simulink model "inv_psm"  (R2026b)
settings: Solver=ode23tb  StopTime=param.sim.simlength  FixedStep=param.sim.tc  MaxStep=param.glb_time.tc
values from neighbouring files (symbols this model uses):
  param = struct()    [init_model.m]
undefined symbols (not defined in the file or in its folder): magnitude
libraries: fl_lib x155, nesl_utility x77, igbt_simple_2th_lib x6, lithium_ion_battery x2, simple_flexible_shaft x2, cstblocks_lti x2, dclink_with_center_tap x1, three_phase_pwm_modulator x1, three_phase_inverter_ideal_switch_based_model x1, three_phase_inverter_igbt_advanced_thermal_model x1, three_phase_inverter_mosfet_based_with_thermal_model x1, threephase_inductor_lib x1
(part 1 of 6)
settings Model: Creator=dbagn  LastModifiedBy=dbagn
settings SolverCC: SolverResetMethod=Robust  ZeroCrossControl=DisableAll
settings DataIOCC: DSMLogging=off  ReturnWorkspaceOutputs=off  SaveOutput=off  SaveTime=off  SignalLogging=off
settings OptimizationCC: ReuseModelBlockBuffer=off
settings SFSimCC: CustomCodeUndefinedFunction=ThrowError  DefaultCustomCodeDeterministicFunctions=All
settings SFSimCC: SimCustomHeaderCode=|
  | #include "rpi.h"
  | #include "mavgflt.h"
  | #include "mavgflt_simulink.h"
  | #include "mavgflts.h"
  | #include "mavgflts_simulink.h"
  | #include "dsmavgflt.h"
  | #include "dsmavgflt_simulink.h"
  | #include "bemf_obsv.h"
  | #include "bemf_obsv_simulink.h"
  | #include "bemf_obsv_load_est.h"
  | #include "bemf_obsv_load_est_simulink.h"
  | #include "dqvector_pi.h"
  | #include "dqvector_pi_simulink.h"
  | #include "sv_pwm_simulink.h"
  | #include "sv_pwm.h"
  | #include "first_harmonic_tracker.h"
  | #include "first_harmonic_tracker_simulink.h"
  | #include "dqpll_thyr.h"
  | #include "dqpll_thyr_simulink.h"
  | #include "dqpll_grid.h"
  | #include "dqpll_grid_simulink.h"
settings SFSimCC: SimUserIncludeDirs=|
  | include
  | src
settings SFSimCC: SimUserSources=|
  | "rpi.c"
  | "mavgflt_simulink.c"
  | "mavgflt.c"
  | "mavgflts_simulink.c"
  | "mavgflts.c"
  | "dsmavgflt_simulink.c"
  | "dsmavgflt.c"
  | "bemf_obsv_simulink.c"
  | "bemf_obsv.c"
  | "bemf_obsv_load_est_simulink.c"
  | "bemf_obsv_load_est.c"
  | "dqvector_pi.c"
  | "dqvector_pi_simulink.c"
  | "sv_pwm_simulink.c"
  | "sv_pwm.c"
  | "first_harmonic_tracker_simulink.c"
  | "first_harmonic_tracker.c"
  | "dqpll_thyr_simulink.c"
  | "dqpll_thyr.c"
  | "dqpll_grid_simulink.c"
  | "dqpll_grid.c"
settings RTWCC: DLArmComputeVersion=19.05
settings SimscapeCC: SimscapeUseEnergyAccounting=off

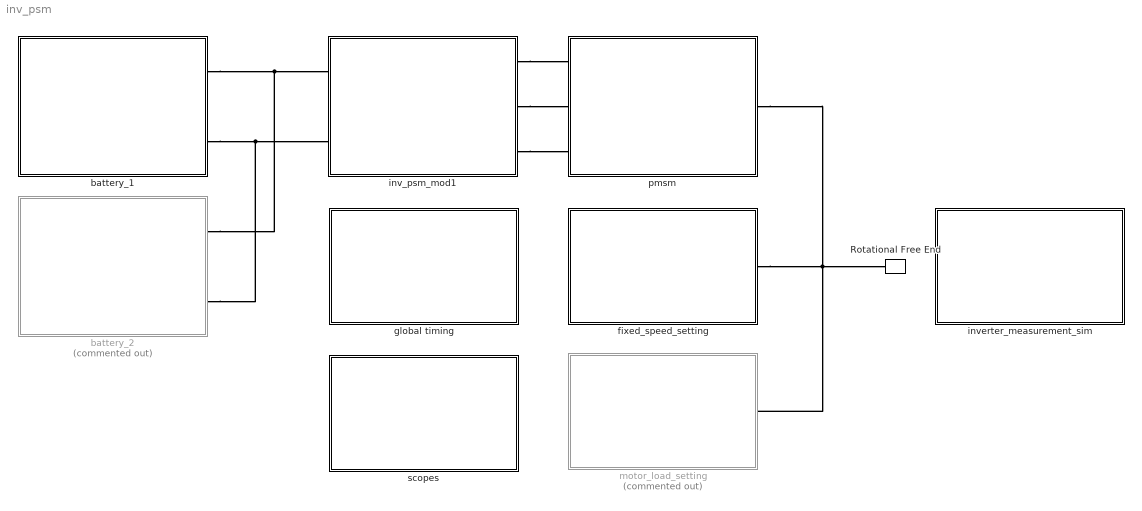
== system inv_psm ==
  Rotational Free End : fl_lib/Mechanical/Rotational Elements/Rotational Free End  w_specify=off  w_priority=None  w=0 rad/s  w_nominal_specify=off  w_nominal_value=1  w_nominal_unit=rad/s
  battery_1 : Subsystem
  battery_2 : Subsystem  Commented=on
  fixed_speed_setting : Subsystem
  global timing : Subsystem
  inv_psm_mod1 : Subsystem
  inverter_measurement_sim : Subsystem
  motor_load_setting : Subsystem  Commented=on
  pmsm : Subsystem
  scopes : Subsystem
  connections:
  pmsm/RConn1 -- Rotational Free End/LConn1 -- fixed_speed_setting/LConn1 -- motor_load_setting/LConn1
  inv_psm_mod1/RConn2 -- pmsm/LConn2
  inv_psm_mod1/RConn1 -- pmsm/LConn1
  inv_psm_mod1/RConn3 -- pmsm/LConn3
  battery_1/RConn1 -- battery_2/RConn1 -- inv_psm_mod1/LConn1
  battery_1/RConn2 -- inv_psm_mod1/LConn2 -- battery_2/RConn2

== system inv_psm/battery_1 ==
  Solver Configuration1 : nesl_utility/Solver Configuration  PhysicalDomain=network_engine_domain  SubClassName=solver  LeftPortType=input  RightPortType=generic  Tones=[]  Harmonics=[]  SimulateNoise=off  Profile=off  UseLocalSampling=off  EnableSwitchedLinearOptims=on  FrequencyDomain=off  UseCCode=off  RelTol=0.001  AbsTol=0.001  MinStep=1e-09  ToWorkspace=off  RevertToSquareIcSolve=off  NumHomotopyIterations=100  PhasorMode=off  PhasorModeNumHarmonics=1  ConsistencySolver=NEWTON_XTOL_AFTER_FTOL  CanonicalOrdering=CANONICAL  OptimizeIntermediates=OPTIMIZED  MulticoreSolverChoice=BACKWARD_EULER  IndexReductionMethod=DerivativeReplacement  DoDC=on  ResidualTolerance=1e-09  ConsistencyTolSource=GLOBAL  ConsistencyAbsTol=0.001  ConsistencyRelTol=0.001  ConsistencyTolFactor=0.001  UseLocalSolver=on  LocalSolverChoice=NE_BACKWARD_EULER_ADVANCER  ResolveIndetEquations=on  FunctionEvalNumThread=1  LocalSolverSampleTime=param.glb_time.tc  DoFixedCost=on  MaxNonlinIter=param.sim.nonlinear_iterations  MaxModeIter=2  ComputeImpulses=off  ImpulseIterations=2  LinearAlgebra=auto  LinearAlgebraNumThread=0  EquationFormulation=NE_TIME_EF  DelaysMemoryBudget=1024  AutomaticFiltering=on  FilteringTimeConstant=0.001  PartitionStorageMethod=AS_NEEDED  PartitionMemoryBudget=1024  PartitionMethod=BALANCED  MultibodyUseLocalSolver=off  MultibodyLocalSolverChoice=ODE1  MultibodyLocalSolverSampleTime=0.001
  litium ion battery 1 : Scope
      settings: ActiveDisplayYMinimum=-166.63080014270002  ActiveDisplayYMaximum=1499.6922306374129  DataLoggingVariableName=ScopeData3
  litium_ion_battery : lithium_ion_battery/lithium_ion_battery  Q=param.battery.pack_1.Q  number_of_cells=param.battery.pack_1.number_of_cells  E_1=param.battery.pack_1.E_1  E0=param.battery.pack_1.E0  E1=param.battery.pack_1.E1  E2=param.battery.pack_1.E2  E3=param.battery.pack_1.E3  Elog=param.battery.pack_1.Elog  R0=param.battery.pack_1.R0  R1=param.battery.pack_1.R1  C1=param.battery.pack_1.C1  M=param.battery.pack_1.M  alpha=param.battery.pack_1.alpha  soc_init=param.battery.pack_1.soc_init  ts_battery=param.glb_time.ts_dab  q1Kalman=param.battery.pack_1.q1Kalman  q2Kalman=param.battery.pack_1.q2Kalman  q3Kalman=param.battery.pack_1.q3Kalman  rKalman=param.battery.pack_1.rKalman  tc=param.glb_time.tc  enable_white_noise_m=0  battery_voltage_init_m=param.battery.nominal_battery_voltage_1
  single_phase_ui_measure : Subsystem
  dc+ : PMIOPort  Side=Right
  dc- : PMIOPort  Port=2  Side=Right
  wires:
  litium_ion_battery/1 -> litium ion battery 1/1
  connections:
  single_phase_ui_measure/LConn2 -- Solver Configuration1/RConn1 -- litium_ion_battery/RConn2
  single_phase_ui_measure/RConn1 -- dc+/RConn1
  litium_ion_battery/RConn1 -- single_phase_ui_measure/LConn1
  dc-/RConn1 -- single_phase_ui_measure/RConn2

== system inv_psm/battery_2 ==
  litium ion battery 2 : Scope
      settings: ActiveDisplayYMinimum=-4779.68523514888  ActiveDisplayYMaximum=38953.418417165572  DataLoggingVariableName=ScopeData3
  litium_ion_battery : lithium_ion_battery/lithium_ion_battery  Q=param.battery.pack_2.Q  number_of_cells=param.battery.pack_2.number_of_cells  E_1=param.battery.pack_2.E_1  E0=param.battery.pack_2.E0  E1=param.battery.pack_2.E1  E2=param.battery.pack_2.E2  E3=param.battery.pack_2.E3  Elog=param.battery.pack_2.Elog  R0=param.battery.pack_2.R0  R1=param.battery.pack_2.R1  C1=param.battery.pack_2.C1  M=param.battery.pack_2.M  alpha=param.battery.pack_2.alpha  soc_init=param.battery.pack_2.soc_init  ts_battery=param.glb_time.ts_dab  q1Kalman=param.battery.pack_2.q1Kalman  q2Kalman=param.battery.pack_2.q2Kalman  q3Kalman=param.battery.pack_2.q3Kalman  rKalman=param.battery.pack_2.rKalman  tc=param.glb_time.tc  enable_white_noise_m=0  battery_voltage_init_m=param.battery.nominal_battery_voltage_1
  single_phase_ui_measure : Subsystem
  dc+ : PMIOPort  Side=Right
  dc- : PMIOPort  Port=2  Side=Right
  wires:
  litium_ion_battery/1 -> litium ion battery 2/1
  connections:
  dc-/RConn1 -- single_phase_ui_measure/RConn2
  litium_ion_battery/RConn1 -- single_phase_ui_measure/LConn1
  single_phase_ui_measure/RConn1 -- dc+/RConn1
  single_phase_ui_measure/LConn2 -- litium_ion_battery/RConn2

== system inv_psm/fixed_speed_setting ==
  Ideal Angular Velocity Source : fl_lib/Mechanical/Mechanical Sources/Ideal Angular Velocity Source
  Mechanical Rotational Reference : fl_lib/Mechanical/Rotational Elements/Mechanical Rotational Reference
  PS Add : fl_lib/Physical Signals/Functions/PS Add
  PS Step1 : fl_lib/Physical Signals/Sources/PS Step  step_time=0.025 s  initial_value=0 rpm  final_value=param.load.rpm_sim rpm
  PS Step2 : fl_lib/Physical Signals/Sources/PS Step  step_time=1.0 s  initial_value=0 rpm  final_value=-2*param.load.rpm_sim rpm
  PS Transfer Function : fl_lib/Physical Signals/Linear Operators/PS Transfer Function  transfer_function_type=foundation.enum.transfer_function_type.lag  T=0.25 s  T1=2 s  T2=1 s  reset_method=foundation.enum.IntegratorResetSpec.None  initial_condition_spec=foundation.enum.IntegratorICSpec.Internal  y0=0 rpm
  flexible_shaft : simple_flexible_shaft/flexible_shaft  Commented=through  b1=1  b2=1  J1=1  J2=1  b_displacement=1e5  k_displacement=1e8
  shaft : PMIOPort  Side=Left
  connections:
  Mechanical Rotational Reference/LConn1 -- Ideal Angular Velocity Source/RConn2
  PS Transfer Function/RConn1 -- Ideal Angular Velocity Source/RConn1
  shaft/RConn1 -- flexible_shaft/LConn1
  flexible_shaft/RConn1 -- Ideal Angular Velocity Source/LConn1
  PS Add/LConn1 -- PS Step1/RConn1
  PS Add/LConn2 -- PS Step2/RConn1
  PS Add/RConn1 -- PS Transfer Function/LConn1

== system inv_psm/global timing ==
  From9 : From  Commented=on  GotoTag=local_time_corr_afe1
  Unit Delay : UnitDelay  SampleTime=param.glb_time.tc
  Unit Delay1 : UnitDelay  SampleTime=param.glb_time.tc
  time_afe1 : Subsystem  mask{k=param.afe.behav.time_gain_module_1}
      mask prompts: k "Time Gain"
      mask Display:
      | disp('time-gen');
      | port_label('input', 1, 'crt');
      | port_label('output', 1, 'tout');
  time_afe3 : Subsystem  mask{k=1}
      mask prompts: k "Time Gain"
      mask Display:
      | disp('time-gen');
      | port_label('output', 1, 'tout');
  time_inv1 : Subsystem  mask{k=param.inv.behav.time_gain_module_2}
      mask prompts: k "Time Gain"
      mask Display:
      | disp('time-gen');
      | port_label('input', 1, 'crt');
      | port_label('output', 1, 'tout');
  tag scope: time_afe_module_1=global, time_inv_module_1=global, time_master=global
  wires:
  time_afe1/1(Out1) -> [time_afe_module_1]
  time_inv1/1(Out1) -> [time_inv_module_1]
  time_afe3/1(Out1) -> [time_master]
  Unit Delay/1 -> time_afe1/1(correction_time)
  Unit Delay1/1 -> time_inv1/1(correction_time)

== system inv_psm/inv_psm_mod1 ==
  dc_source : Subsystem
  inverter : Subsystem
  inverter_ctrl : Subsystem
  output_filter : Subsystem
  us_u : PMIOPort  Side=Right
  us_v : PMIOPort  Port=2  Side=Right
  us_w : PMIOPort  Port=3  Side=Right
  udc(+) : PMIOPort  Port=4  Side=Left
  udc(-) : PMIOPort  Port=5  Side=Left
  wires:
  inverter_ctrl/1(duvw_out) -> inverter/1(duvw)
  connections:
  inverter/LConn2 -- output_filter/RConn2
  inverter/LConn1 -- output_filter/RConn1
  inverter/LConn3 -- output_filter/RConn3
  output_filter/LConn2 -- us_v/RConn1
  output_filter/LConn3 -- us_w/RConn1
  output_filter/LConn1 -- us_u/RConn1
  inverter/RConn1 -- dc_source/RConn1
  inverter/RConn2 -- dc_source/RConn2
  dc_source/LConn2 -- udc(-)/RConn1
  dc_source/LConn1 -- udc(+)/RConn1

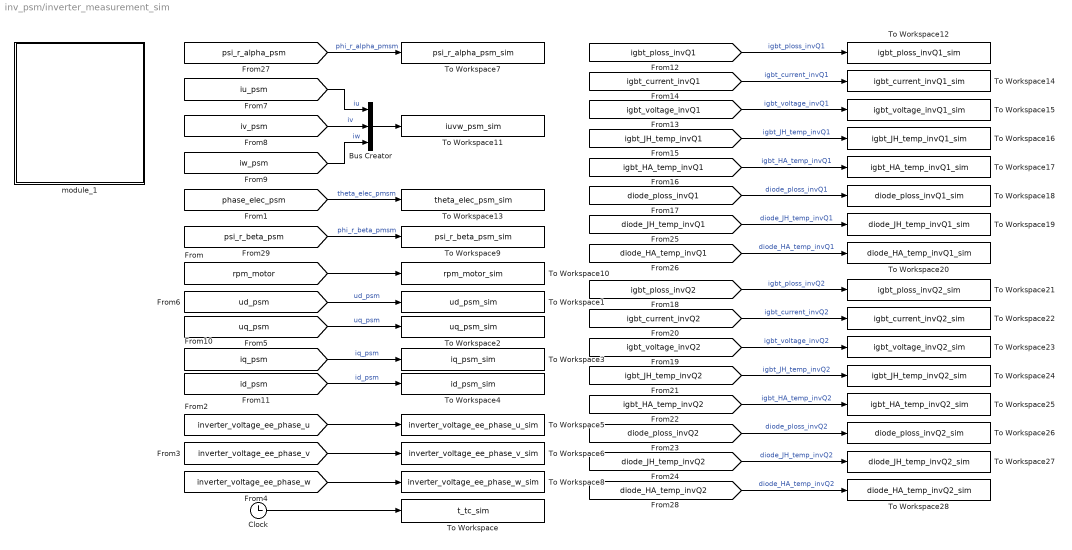
== system inv_psm/inverter_measurement_sim ==
  Bus Creator : BusCreator  Inputs=3
  Clock : Clock
  To Workspace : ToWorkspace  VariableName=t_tc_sim  SampleTime=param.glb_time.tc
      settings: MaxDataPoints=param.glb_time.Nc  Decimation=param.glb_time.decimation_tc
  To Workspace1 : ToWorkspace  VariableName=ud_psm_sim  SampleTime=param.glb_time.tc
      settings: MaxDataPoints=param.glb_time.Nc  Decimation=param.glb_time.decimation_tc
  To Workspace10 : ToWorkspace  VariableName=rpm_motor_sim  SampleTime=param.glb_time.tc
      settings: MaxDataPoints=param.glb_time.Nc  Decimation=param.glb_time.decimation_tc
  To Workspace11 : ToWorkspace  VariableName=iuvw_psm_sim  SampleTime=param.glb_time.tc
      settings: MaxDataPoints=param.glb_time.Nc  Decimation=param.glb_time.decimation_tc
  To Workspace12 : ToWorkspace  VariableName=igbt_ploss_invQ1_sim  SampleTime=param.glb_time.tc
      settings: MaxDataPoints=param.glb_time.Nc  Decimation=param.glb_time.decimation_tc
  To Workspace13 : ToWorkspace  VariableName=theta_elec_psm_sim  SampleTime=param.glb_time.tc
      settings: MaxDataPoints=param.glb_time.Nc  Decimation=param.glb_time.decimation_tc
  To Workspace14 : ToWorkspace  VariableName=igbt_current_invQ1_sim  SampleTime=param.glb_time.tc
      settings: MaxDataPoints=param.glb_time.Nc  Decimation=param.glb_time.decimation_tc
  To Workspace15 : ToWorkspace  VariableName=igbt_voltage_invQ1_sim  SampleTime=param.glb_time.tc
      settings: MaxDataPoints=param.glb_time.Nc  Decimation=param.glb_time.decimation_tc
  To Workspace16 : ToWorkspace  VariableName=igbt_JH_temp_invQ1_sim  SampleTime=param.glb_time.tc
      settings: MaxDataPoints=param.glb_time.Nc  Decimation=param.glb_time.decimation_tc
  To Workspace17 : ToWorkspace  VariableName=igbt_HA_temp_invQ1_sim  SampleTime=param.glb_time.tc
      settings: MaxDataPoints=param.glb_time.Nc  Decimation=param.glb_time.decimation_tc
  To Workspace18 : ToWorkspace  VariableName=diode_ploss_invQ1_sim  SampleTime=param.glb_time.tc
      settings: MaxDataPoints=param.glb_time.Nc  Decimation=param.glb_time.decimation_tc
  To Workspace19 : ToWorkspace  VariableName=diode_JH_temp_invQ1_sim  SampleTime=param.glb_time.tc
      settings: MaxDataPoints=param.glb_time.Nc  Decimation=param.glb_time.decimation_tc
  To Workspace2 : ToWorkspace  VariableName=uq_psm_sim  SampleTime=param.glb_time.tc
      settings: MaxDataPoints=param.glb_time.Nc  Decimation=param.glb_time.decimation_tc
  To Workspace20 : ToWorkspace  VariableName=diode_HA_temp_invQ1_sim  SampleTime=param.glb_time.tc
      settings: MaxDataPoints=param.glb_time.Nc  Decimation=param.glb_time.decimation_tc
  To Workspace21 : ToWorkspace  VariableName=igbt_ploss_invQ2_sim  SampleTime=param.glb_time.tc
      settings: MaxDataPoints=param.glb_time.Nc  Decimation=param.glb_time.decimation_tc
  To Workspace22 : ToWorkspace  VariableName=igbt_current_invQ2_sim  SampleTime=param.glb_time.tc
      settings: MaxDataPoints=param.glb_time.Nc  Decimation=param.glb_time.decimation_tc
  To Workspace23 : ToWorkspace  VariableName=igbt_voltage_invQ2_sim  SampleTime=param.glb_time.tc
      settings: MaxDataPoints=param.glb_time.Nc  Decimation=param.glb_time.decimation_tc
  To Workspace24 : ToWorkspace  VariableName=igbt_JH_temp_invQ2_sim  SampleTime=param.glb_time.tc
      settings: MaxDataPoints=param.glb_time.Nc  Decimation=param.glb_time.decimation_tc
  To Workspace25 : ToWorkspace  VariableName=igbt_HA_temp_invQ2_sim  SampleTime=param.glb_time.tc
      settings: MaxDataPoints=param.glb_time.Nc  Decimation=param.glb_time.decimation_tc
  To Workspace26 : ToWorkspace  VariableName=diode_ploss_invQ2_sim  SampleTime=param.glb_time.tc
      settings: MaxDataPoints=param.glb_time.Nc  Decimation=param.glb_time.decimation_tc
  To Workspace27 : ToWorkspace  VariableName=diode_JH_temp_invQ2_sim  SampleTime=param.glb_time.tc
      settings: MaxDataPoints=param.glb_time.Nc  Decimation=param.glb_time.decimation_tc
  To Workspace28 : ToWorkspace  VariableName=diode_HA_temp_invQ2_sim  SampleTime=param.glb_time.tc
      settings: MaxDataPoints=param.glb_time.Nc  Decimation=param.glb_time.decimation_tc
  To Workspace3 : ToWorkspace  VariableName=iq_psm_sim  SampleTime=param.glb_time.tc
      settings: MaxDataPoints=param.glb_time.Nc  Decimation=param.glb_time.decimation_tc
  To Workspace4 : ToWorkspace  VariableName=id_psm_sim  SampleTime=param.glb_time.tc
      settings: MaxDataPoints=param.glb_time.Nc  Decimation=param.glb_time.decimation_tc
  To Workspace5 : ToWorkspace  VariableName=inverter_voltage_ee_phase_u_sim  SampleTime=param.glb_time.tc
      settings: MaxDataPoints=param.glb_time.Nc  Decimation=param.glb_time.decimation_tc
  To Workspace6 : ToWorkspace  VariableName=inverter_voltage_ee_phase_v_sim  SampleTime=param.glb_time.tc
      settings: MaxDataPoints=param.glb_time.Nc  Decimation=param.glb_time.decimation_tc
  To Workspace7 : ToWorkspace  VariableName=psi_r_alpha_psm_sim  SampleTime=param.glb_time.tc
      settings: MaxDataPoints=param.glb_time.Nc  Decimation=param.glb_time.decimation_tc
  To Workspace8 : ToWorkspace  VariableName=inverter_voltage_ee_phase_w_sim  SampleTime=param.glb_time.tc
      settings: MaxDataPoints=param.glb_time.Nc  Decimation=param.glb_time.decimation_tc
  To Workspace9 : ToWorkspace  VariableName=psi_r_beta_psm_sim  SampleTime=param.glb_time.tc
      settings: MaxDataPoints=param.glb_time.Nc  Decimation=param.glb_time.decimation_tc
  module_1 : Subsystem
  wires:
  [psi_r_alpha_psm] -> To Workspace7/1  "phi_r_alpha_pmsm"
  [psi_r_beta_psm] -> To Workspace9/1  "phi_r_beta_pmsm"
  [rpm_motor] -> To Workspace10/1
  [iv_psm] -> Bus Creator/2  "iv"
  [iw_psm] -> Bus Creator/3  "iw"
  [iu_psm] -> Bus Creator/1  "iu"
  Bus Creator/1 -> To Workspace11/1
  [phase_elec_psm] -> To Workspace13/1  "theta_elec_pmsm"
  [ud_psm] -> To Workspace1/1  "ud_psm"
  [uq_psm] -> To Workspace2/1  "uq_psm"
  [iq_psm] -> To Workspace3/1  "iq_psm"
  [id_psm] -> To Workspace4/1  "id_psm"
  [inverter_voltage_ee_phase_u] -> To Workspace5/1
  [inverter_voltage_ee_phase_v] -> To Workspace6/1
  [inverter_voltage_ee_phase_w] -> To Workspace8/1
  [diode_HA_temp_invQ1] -> To Workspace20/1  "diode_HA_temp_invQ1"
  [igbt_current_invQ1] -> To Workspace14/1  "igbt_current_invQ1"
  [diode_ploss_invQ1] -> To Workspace18/1  "diode_ploss_invQ1"
  [diode_JH_temp_invQ1] -> To Workspace19/1  "diode_JH_temp_invQ1"
  [igbt_HA_temp_invQ1] -> To Workspace17/1  "igbt_HA_temp_invQ1"
  [igbt_ploss_invQ1] -> To Workspace12/1  "igbt_ploss_invQ1"
  [igbt_voltage_invQ1] -> To Workspace15/1  "igbt_voltage_invQ1"
  [igbt_JH_temp_invQ1] -> To Workspace16/1  "igbt_JH_temp_invQ1"
  Clock/1 -> To Workspace/1
  [igbt_JH_temp_invQ2] -> To Workspace24/1  "igbt_JH_temp_invQ2"
  [igbt_voltage_invQ2] -> To Workspace23/1  "igbt_voltage_invQ2"
  [igbt_ploss_invQ2] -> To Workspace21/1  "igbt_ploss_invQ2"
  [igbt_HA_temp_invQ2] -> To Workspace25/1  "igbt_HA_temp_invQ2"
  [diode_JH_temp_invQ2] -> To Workspace27/1  "diode_JH_temp_invQ2"
  [diode_ploss_invQ2] -> To Workspace26/1  "diode_ploss_invQ2"
  [igbt_current_invQ2] -> To Workspace22/1  "igbt_current_invQ2"
  [diode_HA_temp_invQ2] -> To Workspace28/1  "diode_HA_temp_invQ2"

== system inv_psm/motor_load_setting ==
  Ideal Torque Source : fl_lib/Mechanical/Mechanical Sources/Ideal Torque Source
  Inertia : fl_lib/Mechanical/Rotational Elements/Inertia  inertia=param.load.external_load_inertia kg*m^2  num_ports=foundation.enum.numPorts2.one  w_specify=off  w_priority=High  w=0 rad/s  w_nominal_specify=off  w_nominal_value=1  w_nominal_unit=rad/s  t_specify=off  t_priority=None  t=0 N*m  t_nominal_specify=off  t_nominal_value=1  t_nominal_unit=N*m
  Mechanical Rotational Reference : fl_lib/Mechanical/Rotational Elements/Mechanical Rotational Reference
  PS Step : fl_lib/Physical Signals/Sources/PS Step  step_time=param.sim.load_step_time s  initial_value=1 N*m  final_value=1 N*m
  PS Transfer Function : fl_lib/Physical Signals/Linear Operators/PS Transfer Function  transfer_function_type=foundation.enum.transfer_function_type.lag  T=1 s  T1=2 s  T2=1 s  reset_method=foundation.enum.IntegratorResetSpec.None  initial_condition_spec=foundation.enum.IntegratorICSpec.Internal  y0=0 N*m
  flexible_shaft : simple_flexible_shaft/flexible_shaft  b1=1  b2=1  J1=1  J2=1  b_displacement=1  k_displacement=1e5
  shaft : PMIOPort  Side=Left
  connections:
  Ideal Torque Source/LConn1 -- flexible_shaft/RConn1 -- Inertia/LConn1
  Ideal Torque Source/RConn2 -- Mechanical Rotational Reference/LConn1
  PS Transfer Function/RConn1 -- Ideal Torque Source/RConn1
  PS Step/RConn1 -- PS Transfer Function/LConn1
  flexible_shaft/LConn1 -- shaft/RConn1

== system inv_psm/pmsm ==
  Bus Selector1 : BusSelector  OutputSignals=omega_mech (rpm)
  Constant : Constant  Value=param.psm.machine.psi_m
  Simulink-PS Converter3 : nesl_utility/Simulink-PS Converter  PhysicalDomain=network_engine_domain  SubClassName=ps_input  LeftPortType=input  RightPortType=output  PseudoPeriodic=off  Frequencies=[]  NoiseDistribution=none  NoiseParameters=[]  Unit=V*s  AffineConversion=on  FilteringAndDerivatives=provide  SimscapeFilterOrder=1  InputFilterTimeConstant=0.001  UdotUserProvided=0
  synchronous_motor : Subsystem
  u : PMIOPort  Side=Left
  v : PMIOPort  Port=2  Side=Left
  w : PMIOPort  Port=3  Side=Left
  shaft : PMIOPort  Port=4  Side=Right
  tag scope: rpm_motor=global
  wires:
  synchronous_motor/1(motor_data) -> Bus Selector1/1
  Bus Selector1/1 -> [rpm_motor]  "<omega_mech (rpm)>"
  Constant/1 -> Simulink-PS Converter3/1
  connections:
  synchronous_motor/LConn1 -- u/RConn1
  Simulink-PS Converter3/RConn1 -- synchronous_motor/LConn4
  synchronous_motor/LConn3 -- w/RConn1
  synchronous_motor/LConn2 -- v/RConn1
  shaft/RConn1 -- synchronous_motor/RConn1

== system inv_psm/scopes ==
  igbt_losses : Subsystem
  inverter_data : Subsystem
  power_mosfet_losses : Subsystem  Commented=on

== system inv_psm/battery_1/single_phase_ui_measure ==
  Bus Creator : BusCreator  Inputs=2
  Current Sensor : fl_lib/Electrical/Electrical Sensors/Current Sensor
  Selector : Selector  InputPortWidth=2  IndexOptions=Index vector (dialog)  Indices=2  OutputSizes=1  RuntimeRangeChecks=off
  Selector1 : Selector  InputPortWidth=2  IndexOptions=Index vector (dialog)  Indices=1  OutputSizes=1  RuntimeRangeChecks=off
  Voltage Sensor : fl_lib/Electrical/Electrical Sensors/Voltage Sensor
  dab input modA : Scope  NumInputPorts=2
      settings: SampleTime=param.glb_time.tc  ActiveDisplayYMinimum=0.016673817947882516  ActiveDisplayYMaximum=0.038331642126922673  DataLoggingVariableName=ScopeData2
  iph : nesl_utility/PS-Simulink Converter  PhysicalDomain=network_engine_domain  SubClassName=ps_output  LeftPortType=input  RightPortType=output  PseudoPeriodic=off  Frequencies=[]  VectorFormat=1-D array  Unit=A  AffineConversion=off
  uph : nesl_utility/PS-Simulink Converter  PhysicalDomain=network_engine_domain  SubClassName=ps_output  LeftPortType=input  RightPortType=output  PseudoPeriodic=off  Frequencies=[]  VectorFormat=1-D array  Unit=V  AffineConversion=off
  Udc(+) : PMIOPort  Side=Left
  udc(+) : PMIOPort  Port=2  Side=Right
  Udc(-) : PMIOPort  Port=3  Side=Left
  udc(-) : PMIOPort  Port=4  Side=Right
  tag scope: current_battery_1=global, voltage_battery_1=global
  wires:
  Bus Creator/1 -> Selector/1, Selector1/1  "ui_data"
  iph/1 -> Bus Creator/1  "iph"
  uph/1 -> Bus Creator/2  "uph"
  Selector1/1 -> [current_battery_1], dab input modA/1  "current_battery"
  Selector/1 -> dab input modA/2, [voltage_battery_1]  "voltage_battery"
  connections:
  iph/LConn1 -- Current Sensor/RConn1
  Voltage Sensor/LConn1 -- Current Sensor/LConn1 -- Udc(+)/RConn1
  Current Sensor/RConn2 -- udc(+)/RConn1
  Voltage Sensor/RConn1 -- uph/LConn1
  Voltage Sensor/RConn2 -- Udc(-)/RConn1 -- udc(-)/RConn1

== system inv_psm/battery_2/single_phase_ui_measure ==
  Bus Creator : BusCreator  Inputs=2
  Current Sensor : fl_lib/Electrical/Electrical Sensors/Current Sensor
  Selector : Selector  InputPortWidth=2  IndexOptions=Index vector (dialog)  Indices=2  OutputSizes=1  RuntimeRangeChecks=off
  Selector1 : Selector  InputPortWidth=2  IndexOptions=Index vector (dialog)  Indices=1  OutputSizes=1  RuntimeRangeChecks=off
  Voltage Sensor : fl_lib/Electrical/Electrical Sensors/Voltage Sensor
  dab input modA : Scope  NumInputPorts=2
      settings: SampleTime=param.glb_time.tc  ActiveDisplayYMinimum=-363.9315036867377  ActiveDisplayYMaximum=456.02820990604641  DataLoggingVariableName=ScopeData2
  iph : nesl_utility/PS-Simulink Converter  PhysicalDomain=network_engine_domain  SubClassName=ps_output  LeftPortType=input  RightPortType=output  PseudoPeriodic=off  Frequencies=[]  VectorFormat=1-D array  Unit=A  AffineConversion=off
  uph : nesl_utility/PS-Simulink Converter  PhysicalDomain=network_engine_domain  SubClassName=ps_output  LeftPortType=input  RightPortType=output  PseudoPeriodic=off  Frequencies=[]  VectorFormat=1-D array  Unit=V  AffineConversion=off
  Udc(+) : PMIOPort  Side=Left
  udc(+) : PMIOPort  Port=2  Side=Right
  Udc(-) : PMIOPort  Port=3  Side=Left
  udc(-) : PMIOPort  Port=4  Side=Right
  tag scope: current_battery_2=global, voltage_battery_2=global
  wires:
  Selector/1 -> [voltage_battery_2], dab input modA/2  "voltage_battery"
  Selector1/1 -> dab input modA/1, [current_battery_2]  "current_battery"
  uph/1 -> Bus Creator/2  "uph"
  iph/1 -> Bus Creator/1  "iph"
  Bus Creator/1 -> Selector1/1, Selector/1  "ui_data"
  connections:
  udc(-)/RConn1 -- Udc(-)/RConn1 -- Voltage Sensor/RConn2
  Voltage Sensor/RConn1 -- uph/LConn1
  Current Sensor/RConn2 -- udc(+)/RConn1
  Udc(+)/RConn1 -- Current Sensor/LConn1 -- Voltage Sensor/LConn1
  iph/LConn1 -- Current Sensor/RConn1

== system inv_psm/global timing/time_afe1 ==
  correction_time : Inport
  Constant : Constant
  Gain : Gain  Gain=k
  Product : Product
  Sum : Sum  Inputs=|++
  time_1 : Clock
  Out1 : Outport
  wires:
  time_1/1 -> Gain/1
  Gain/1 -> Product/1
  Product/1 -> Out1/1
  correction_time/1 -> Sum/1
  Sum/1 -> Product/2
  Constant/1 -> Sum/2

== system inv_psm/global timing/time_afe3 ==
  Gain : Gain  Gain=k
  time_1 : Clock
  Out1 : Outport
  wires:
  Gain/1 -> Out1/1
  time_1/1 -> Gain/1

== system inv_psm/global timing/time_inv1 ==
  correction_time : Inport
  Constant : Constant
  Gain : Gain  Gain=k
  Product : Product
  Sum : Sum  Inputs=|++
  time_1 : Clock
  Out1 : Outport
  wires:
  time_1/1 -> Gain/1
  Gain/1 -> Product/1
  Product/1 -> Out1/1
  correction_time/1 -> Sum/1
  Constant/1 -> Sum/2
  Sum/1 -> Product/2

== system inv_psm/inv_psm_mod1/dc_source ==
  Bus Selector : BusSelector  OutputSignals=udc,Cdc1_current,vdc_pu
  Electrical Reference : fl_lib/Electrical/Electrical Elements/Electrical Reference
  dclink : dclink_with_center_tap/dclink  Cdc1=param.inv.hw.CFi1  Cdc2=param.inv.hw.CFi2  Rudc_measure=param.inv.hw.Rudc_measure  Vdc_scale=param.battery.pack_1.Vbattery_nom
  udc(+) : PMIOPort  Side=Right
  udc(-) : PMIOPort  Port=2  Side=Right
  Udc(+) : PMIOPort  Port=3  Side=Left
  Udc(-) : PMIOPort  Port=4  Side=Left
  tag scope: all_voltages_about_dclink=global, ic_dclink_mod1=global, udc_mod1=global, vdc_pu_inv_mod1=global
  wires:
  dclink/1 -> Bus Selector/1, [all_voltages_about_dclink]
  Bus Selector/1 -> [udc_mod1]  "<udc>"
  Bus Selector/2 -> [ic_dclink_mod1]  "<Cdc1_current>"
  Bus Selector/3 -> [vdc_pu_inv_mod1]  "<vdc_pu>"
  connections:
  dclink/LConn1 -- udc(+)/RConn1
  udc(-)/RConn1 -- dclink/LConn2
  dclink/RConn3 -- Udc(-)/RConn1
  dclink/RConn1 -- Udc(+)/RConn1
  dclink/RConn2 -- Electrical Reference/LConn1

== system inv_psm/inv_psm_mod1/inverter ==
  duvw : Inport
  Current Sensor : fl_lib/Electrical/Electrical Sensors/Current Sensor
  PS-Simulink Converter1 : nesl_utility/PS-Simulink Converter  PhysicalDomain=network_engine_domain  SubClassName=ps_output  LeftPortType=input  RightPortType=output  PseudoPeriodic=off  Frequencies=[]  VectorFormat=1-D array  Unit=A  AffineConversion=on
  PS-Simulink Converter4 : nesl_utility/PS-Simulink Converter  PhysicalDomain=network_engine_domain  SubClassName=ps_output  LeftPortType=input  RightPortType=output  PseudoPeriodic=off  Frequencies=[]  VectorFormat=1-D array  Unit=V  AffineConversion=on
  To Workspace : ToWorkspace  VariableName=idc_sim_mod1  SampleTime=param.glb_time.tc
      settings: MaxDataPoints=param.glb_time.Nc
  To Workspace1 : ToWorkspace  VariableName=udc_sim_mod1  SampleTime=param.glb_time.tc
      settings: MaxDataPoints=param.glb_time.Nc
  Transfer Fcn : TransferFcn  Denominator=[1e-2 1]
  Voltage Sensor : fl_lib/Electrical/Electrical Sensors/Voltage Sensor
  idc/udc : Scope  NumInputPorts=2
      settings: SampleTime=param.glb_time.tc  ActiveDisplayYMinimum=-232.79227304961765  ActiveDisplayYMaximum=27.545875945686063
  inverter : Subsystem
  Udc(+) : PMIOPort  Side=Right
  Udc(-) : PMIOPort  Port=2  Side=Right
  us_u : PMIOPort  Port=3  Side=Left
  us_v : PMIOPort  Port=4  Side=Left
  us_w : PMIOPort  Port=5  Side=Left
  wires:
  PS-Simulink Converter4/1 -> To Workspace1/1, idc/udc/2  "udc"
  PS-Simulink Converter1/1 -> Transfer Fcn/1  "idc"
  Transfer Fcn/1 -> To Workspace/1, idc/udc/1  "idc_flt"
  duvw/1 -> inverter/1(gate_cmds_uvw)
  connections:
  PS-Simulink Converter4/LConn1 -- Voltage Sensor/RConn1
  us_u/RConn1 -- inverter/LConn1
  us_v/RConn1 -- inverter/LConn2
  us_w/RConn1 -- inverter/LConn3
  Voltage Sensor/RConn2 -- inverter/RConn2 -- Udc(-)/RConn1
  Current Sensor/LConn1 -- Udc(+)/RConn1
  Voltage Sensor/LConn1 -- inverter/RConn1 -- Current Sensor/RConn2
  PS-Simulink Converter1/LConn1 -- Current Sensor/RConn1

== system inv_psm/inv_psm_mod1/inverter_ctrl ==
  inverter_control : Subsystem
  duvw_out : Outport
  tag scope: local_time_corr_inv1=global, master_torque_ref=global
  wires:
  [is_uvw_pu_mod1] -> inverter_control/1(is_uvw)
  [TRGO_inv_module_1] -> inverter_control/Trigger
  [vdc_pu_inv_mod1] -> inverter_control/2(udc_pu)
  inverter_control/1(duvw) -> duvw_out/1
  [time_inv_module_1] -> inverter_control/3(local_time)
  [time_master] -> inverter_control/4(master_time)
  inverter_control/2(local_time_corr) -> [local_time_corr_inv1]
  inverter_control/3(master_torque_ref) -> [master_torque_ref]
  [phase_elec_psm] -> inverter_control/5(phase_elec_psm)
  [omega_elec_psm] -> inverter_control/6(omega_elec_psm)

== system inv_psm/inv_psm_mod1/output_filter ==
  Inductor{,1..5} (6 alike) : fl_lib/Electrical/Electrical Elements/Inductor  l=1e-6 H  r=0 Ohm  g=1e-9 1/Ohm  i_specify=off  i_priority=None  i=0 A  i_nominal_specify=off  i_nominal_value=1  i_nominal_unit=A  v_specify=off  v_priority=None  v=0 V  v_nominal_specify=off  v_nominal_value=1  v_nominal_unit=V  i_L_specify=off  i_L_priority=High  i_L=0 A  i_L_nominal_specify=off  i_L_nominal_value=1  i_L_nominal_unit=A
  threephase inductor : threephase_inductor_lib/threephase inductor  Lp=param.inv.hw.LFi H  L0=param.inv.hw.LFi_cm H  Rp=param.inv.hw.RLFi Ohm  R0=param.inv.hw.RLFi_cm Ohm  Lls=5e-6 H  uu_1_specify=off  uu_1_priority=None  uu_1=0 V  uu_1_nominal_specify=off  uu_1_nominal_value=1  uu_1_nominal_unit=V  uv_1_specify=off  uv_1_priority=None  uv_1=0 V  uv_1_nominal_specify=off  uv_1_nominal_value=1  uv_1_nominal_unit=V  uw_1_specify=off  uw_1_priority=None  uw_1=0 V  uw_1_nominal_specify=off  uw_1_nominal_value=1  uw_1_nominal_unit=V  uu_2_specify=off  uu_2_priority=None  uu_2=0 V  uu_2_nominal_specify=off  uu_2_nominal_value=1  uu_2_nominal_unit=V  uv_2_specify=off  uv_2_priority=None  uv_2=0 V  uv_2_nominal_specify=off  uv_2_nominal_value=1  uv_2_nominal_unit=V  uw_2_specify=off  uw_2_priority=None  uw_2=0 V  uw_2_nominal_specify=off  uw_2_nominal_value=1  uw_2_nominal_unit=V  iu_specify=off  iu_priority=None  iu=0 A  iu_nominal_specify=off  iu_nominal_value=1  iu_nominal_unit=A  iv_specify=off  iv_priority=None  iv=0 A  iv_nominal_specify=off  iv_nominal_value=1  iv_nominal_unit=A  iw_specify=off  iw_priority=None  iw=0 A  iw_nominal_specify=off  iw_nominal_value=1  iw_nominal_unit=A
  threephase_vi_measures_stack : Subsystem
  us_u : PMIOPort  Side=Left
  uu : PMIOPort  Port=2  Side=Right
  us_v : PMIOPort  Port=3  Side=Left
  uv : PMIOPort  Port=4  Side=Right
  us_w : PMIOPort  Port=5  Side=Left
  uw : PMIOPort  Port=6  Side=Right
  connections:
  threephase_vi_measures_stack/LConn1 -- us_u/RConn1
  threephase_vi_measures_stack/LConn2 -- us_v/RConn1
  threephase_vi_measures_stack/LConn3 -- us_w/RConn1
  Inductor3/LConn1 -- threephase_vi_measures_stack/RConn1
  threephase inductor/LConn2 -- Inductor4/RConn1
  threephase inductor/LConn3 -- Inductor5/RConn1
  threephase inductor/RConn1 -- Inductor/LConn1
  threephase inductor/RConn2 -- Inductor1/LConn1
  threephase inductor/RConn3 -- Inductor2/LConn1
  Inductor/RConn1 -- uu/RConn1
  Inductor1/RConn1 -- uv/RConn1
  Inductor2/RConn1 -- uw/RConn1
  threephase inductor/LConn1 -- Inductor3/RConn1
  Inductor4/LConn1 -- threephase_vi_measures_stack/RConn2
  Inductor5/LConn1 -- threephase_vi_measures_stack/RConn3

== system inv_psm/inverter_measurement_sim/module_1 ==
  From6 : From  Commented=on  GotoTag=ileg_dc_inv_mod1
  To Workspace12 : ToWorkspace  Commented=on  VariableName=ileg_dc_inv_sim_mod1  SampleTime=param.glb_time.tc
      settings: MaxDataPoints=param.glb_time.Nc  Decimation=param.glb_time.decimation_tc
  To Workspace14 : ToWorkspace  VariableName=is_uvw_sim_mod1  SampleTime=param.glb_time.tc
      settings: MaxDataPoints=param.glb_time.Nc  Decimation=param.glb_time.decimation_tc
  To Workspace15 : ToWorkspace  VariableName=us_uvw_sim_mod1  SampleTime=param.glb_time.tc
      settings: MaxDataPoints=param.glb_time.Nc  Decimation=param.glb_time.decimation_tc
  wires:
  [us_uvw_pu_mod1] -> To Workspace15/1
  From6/1 -> To Workspace12/1
  [is_uvw_pu_mod1] -> To Workspace14/1

== system inv_psm/pmsm/synchronous_motor ==
  Bus Selector : BusSelector  OutputSignals=psi_r_alpha (Vs)
  Bus Selector1 : BusSelector  OutputSignals=psi_r_alpha (Vs)
  Bus Selector10 : BusSelector  OutputSignals=uq (V)
  Bus Selector11 : BusSelector  OutputSignals=ud (V)
  Bus Selector12 : BusSelector  OutputSignals=iq (A)
  Bus Selector13 : BusSelector  OutputSignals=id (A)
  Bus Selector2 : BusSelector  OutputSignals=iu (A)
  Bus Selector3 : BusSelector  OutputSignals=iv (A)
  Bus Selector4 : BusSelector  OutputSignals=iw (A)
  Bus Selector5 : BusSelector  OutputSignals=omega_elec (rad/s)
  Bus Selector6 : BusSelector  OutputSignals=phase_elec (rad)
  Bus Selector7 : BusSelector  OutputSignals=pwr_in (kW)
  Bus Selector8 : BusSelector  OutputSignals=pwr_out (kW)
  Bus Selector9 : BusSelector  OutputSignals=torque (Nm)
  Open Circuit : fl_lib/Electrical/Electrical Elements/Open Circuit  v_specify=off  v_priority=None  v=0 V  v_nominal_specify=off  v_nominal_value=1  v_nominal_unit=V
  permanent_magnet_synchronous_machine : permanent_magnet_synchronous_machine/permanent_magnet_synchronous_machine  pp=param.psm.machine.number_poles  psi_m=param.psm.machine.psi_m  Lmu=param.psm.machine.Lmu  La=param.psm.machine.La_m  Lb=param.psm.machine.Lb_m  Rs=param.psm.machine.Rs_m  Jm=param.psm.machine.Jm_m  b_linear=param.psm.machine.load_friction_m  b_quadratic=0  h5_percent=0  h7_percent=0  psi_r_u_init=param.psm.machine.psi_m  psi_r_v_init=-param.psm.machine.psi_m/2  psi_r_w_init=-param.psm.machine.psi_m/2  omega_init=0  phase_init=0  angle_error=0
  shaft : PMIOPort  Side=Right
  u : PMIOPort  Port=2  Side=Left
  v : PMIOPort  Port=3  Side=Left
  w : PMIOPort  Port=4  Side=Left
  psi_m : PMIOPort  Port=5  Side=Left
  motor_data : Outport
  tag scope: id_psm=global, iq_psm=global, iu_psm=global, iv_psm=global, iw_psm=global, omega_elec_psm=global, phase_elec_psm=global, psi_r_alpha_psm=global, psi_r_beta_psm=global, pwr_in_psm=global, pwr_out_psm=global, torque_load_psm=global, ud_psm=global, uq_psm=global
  wires:
  permanent_magnet_synchronous_machine/1 -> Bus Selector8/1, Bus Selector10/1, Bus Selector11/1, Bus Selector12/1, Bus Selector13/1, Bus Selector9/1, Bus Selector7/1, Bus Selector6/1, Bus Selector5/1, Bus Selector4/1, Bus Selector3/1, Bus Selector2/1, Bus Selector1/1, Bus Selector/1, motor_data/1
  Bus Selector/1 -> [psi_r_alpha_psm]  "<psi_r_alpha (Vs)>"
  Bus Selector1/1 -> [psi_r_beta_psm]  "<psi_r_alpha (Vs)>"
  Bus Selector2/1 -> [iu_psm]  "<iu (A)>"
  Bus Selector3/1 -> [iv_psm]  "<iv (A)>"
  Bus Selector4/1 -> [iw_psm]  "<iw (A)>"
  Bus Selector5/1 -> [omega_elec_psm]  "<omega_elec (rad/s)>"
  Bus Selector6/1 -> [phase_elec_psm]  "<phase_elec (rad)>"
  Bus Selector7/1 -> [pwr_in_psm]  "<pwr_in (kW)>"
  Bus Selector8/1 -> [pwr_out_psm]  "<pwr_out (kW)>"
  Bus Selector9/1 -> [torque_load_psm]  "<torque (Nm)>"
  Bus Selector10/1 -> [uq_psm]  "<uq (V)>"
  Bus Selector11/1 -> [ud_psm]  "<ud (V)>"
  Bus Selector12/1 -> [iq_psm]  "<iq (A)>"
  Bus Selector13/1 -> [id_psm]  "<id (A)>"
  connections:
  permanent_magnet_synchronous_machine/RConn1 -- shaft/RConn1
  permanent_magnet_synchronous_machine/LConn1 -- u/RConn1
  permanent_magnet_synchronous_machine/LConn2 -- v/RConn1
  permanent_magnet_synchronous_machine/LConn3 -- w/RConn1
  permanent_magnet_synchronous_machine/LConn4 -- psi_m/RConn1
  permanent_magnet_synchronous_machine/LConn5 -- Open Circuit/LConn1

== system inv_psm/scopes/igbt_losses ==
  Bus Creator10 : BusCreator  Inputs=2
  Bus Creator2 : BusCreator  Inputs=2
  Bus Creator7 : BusCreator  Inputs=2
  diode power losses INV Q1 : Scope  NumInputPorts=2
      settings: SampleTime=param.glb_time.tc  ActiveDisplayYMinimum=-3.7723788379286622  ActiveDisplayYMaximum=34.127063082184456  DataLoggingVariableName=ScopeData31
  igbt power losses INV Q1 : Scope  NumInputPorts=4
      settings: SampleTime=param.glb_time.tc  ActiveDisplayYMinimum=-96.444657981702733  ActiveDisplayYMaximum=880.27949068498833  DataLoggingVariableName=ScopeData16
  igbt power losses INV Q2 : Scope  NumInputPorts=4
      settings: SampleTime=param.glb_time.tc  ActiveDisplayYMinimum=-465.31550512642031  ActiveDisplayYMaximum=483.0191874445743  DataLoggingVariableName=ScopeData27
  wires:
  Bus Creator7/1 -> igbt power losses INV Q2/4
  [igbt_voltage_invQ2] -> igbt power losses INV Q2/3  "igbt_voltage_invQ2"
  [igbt_current_invQ2] -> igbt power losses INV Q2/2  "igbt_current_invQ2"
  [igbt_ploss_invQ2] -> igbt power losses INV Q2/1  "igbt_ploss_invQ2"
  [igbt_JH_temp_invQ2] -> Bus Creator7/1  "igbt_JH_temp_invQ2"
  [igbt_HA_temp_invQ2] -> Bus Creator7/2  "igbt_HA_temp_invQ2"
  [igbt_voltage_invQ1] -> igbt power losses INV Q1/3  "igbt_voltage_invQ1"
  [igbt_JH_temp_invQ1] -> Bus Creator2/1  "igbt_JH_temp_invQ1"
  [diode_JH_temp_invQ1] -> Bus Creator10/1  "diode_JH_temp_invQ1"
  [igbt_current_invQ1] -> igbt power losses INV Q1/2  "igbt_current_invQ1"
  [igbt_HA_temp_invQ1] -> Bus Creator2/2  "igbt_HA_temp_invQ1"
  [diode_HA_temp_invQ1] -> Bus Creator10/2  "diode_HA_temp_invQ1"
  [igbt_ploss_invQ1] -> igbt power losses INV Q1/1  "igbt_ploss_invQ1"
  Bus Creator10/1 -> diode power losses INV Q1/2
  Bus Creator2/1 -> igbt power losses INV Q1/4
  [diode_ploss_invQ1] -> diode power losses INV Q1/1  "diode_ploss_invQ1"

== system inv_psm/scopes/inverter_data ==
  Bus Creator3 : BusCreator  Inputs=2
  Bus Creator4 : BusCreator  Inputs=2
  Bus Creator5 : BusCreator  Inputs=2
  Gain1 : Gain  Gain=1e-3
  LTI System : cstblocks_lti/LTI System  sys=param.ctrl.filters.inv.SOF_50Hz.ss_c  IC=[]  PadeOrder=0
  LTI System1 : cstblocks_lti/LTI System  sys=param.ctrl.filters.inv.SOF_50Hz.ss_c  IC=[]  PadeOrder=0
  idc/udc : Scope  NumInputPorts=2
      settings: SampleTime=param.glb_time.tc  ActiveDisplayYMinimum=-112.73258117348806  ActiveDisplayYMaximum=100.39151113913991  DataLoggingVariableName=ScopeData23
  inverter_voltage_ee : Scope  NumInputPorts=3
      settings: ActiveDisplayYMinimum=-207.5782073641667  ActiveDisplayYMaximum=1301.7632755987056  DataLoggingVariableName=ScopeData30
  is_uvw/us_uvw : Scope  NumInputPorts=2
      settings: SampleTime=param.glb_time.tc  ActiveDisplayYMinimum=-0.9328378987725684  ActiveDisplayYMaximum=0.91243157073040826  DataLoggingVariableName=ScopeData25
  motor currents : Scope  NumInputPorts=3
      settings: SampleTime=param.glb_time.tc  ActiveDisplayYMinimum=429.93806644608685  ActiveDisplayYMaximum=486.36568218837249  DataLoggingVariableName=ScopeData17
  motor dq : Scope  NumInputPorts=2
      settings: SampleTime=param.glb_time.tc  ActiveDisplayYMinimum=-850.02239826316088  ActiveDisplayYMaximum=207.16586596148719  DataLoggingVariableName=ScopeData18
  motor mech : Scope  NumInputPorts=3
      settings: SampleTime=param.glb_time.tc  ActiveDisplayYMinimum=-20.999581204315788  ActiveDisplayYMaximum=21.716285550669411  DataLoggingVariableName=ScopeData11
  phi_alpha_pmsm/phi_beta_pmsm : Scope  NumInputPorts=2
      settings: SampleTime=param.glb_time.tc  ActiveDisplayYMinimum=-8970.3778212698689  ActiveDisplayYMaximum=-8969.2326513408079  DataLoggingVariableName=ScopeData19
  udc voltages : Scope  NumInputPorts=2
      settings: SampleTime=param.glb_time.tc  ActiveDisplayYMinimum=1.0380539759820944  ActiveDisplayYMaximum=1.0407256681154484  DataLoggingVariableName=ScopeData24
  wires:
  [iv_psm] -> motor currents/2  "iv_psm"
  [id_psm] -> Bus Creator4/2  "id_psm"
  [psi_r_beta_psm] -> phi_alpha_pmsm/phi_beta_pmsm/2
  [iw_psm] -> motor currents/3  "iw_psm"
  [us_uvw_pu_mod1] -> is_uvw/us_uvw/2  "us_uvw_pu_mod1"
  [vdc_pu_inv_mod1] -> udc voltages/1  "udc"
  [torque_load_psm] -> Gain1/1
  [iu_psm] -> motor currents/1  "iu_psm"
  [iq_psm] -> Bus Creator4/1  "iq_psm"
  [is_uvw_pu_mod1] -> is_uvw/us_uvw/1  "is_uvw_pu_mod1"
  [pwr_in_psm] -> LTI System/1
  [all_voltages_about_dclink] -> udc voltages/2  "all_voltages_about_dclink"
  Bus Creator5/1 -> motor mech/3
  [ud_psm] -> Bus Creator3/1  "ud_psm"
  Bus Creator3/1 -> motor dq/1
  [inverter_voltage_ee_phase_w] -> inverter_voltage_ee/3  "inverter_voltage_ee_phase_w"
  LTI System/1 -> Bus Creator5/1  "pin_psm (kW)"
  [pwr_out_psm] -> LTI System1/1
  [rpm_motor] -> motor mech/1  "omega_elec_psm (rpm)"
  Bus Creator4/1 -> motor dq/2
  [inverter_voltage_ee_phase_v] -> inverter_voltage_ee/2  "inverter_voltage_ee_phase_v"
  [inverter_voltage_ee_phase_u] -> inverter_voltage_ee/1  "inverter_voltage_ee_phase_u"
  LTI System1/1 -> Bus Creator5/2  "pwr_out_psm (kW)"
  Gain1/1 -> motor mech/2  "torque_load_psm (kNm)"
  [udc_mod1] -> idc/udc/2  "udc_dclink_mod1"
  [ic_dclink_mod1] -> idc/udc/1  "ic_dclink_mod1"
  [psi_r_alpha_psm] -> phi_alpha_pmsm/phi_beta_pmsm/1
  [uq_psm] -> Bus Creator3/2  "uq_psm"

== system inv_psm/scopes/power_mosfet_losses ==
  Bus Creator8 : BusCreator  Inputs=2
  Bus Creator9 : BusCreator  Inputs=2
  mosfet power losses INV Q1 : Scope  NumInputPorts=4
      settings: SampleTime=param.glb_time.tc  ActiveDisplayYMinimum=-52.647210306071649  ActiveDisplayYMaximum=473.81757031333393  DataLoggingVariableName=ScopeData28
  mosfet power losses INV Q2 : Scope  NumInputPorts=4
      settings: SampleTime=param.glb_time.tc  ActiveDisplayYMinimum=-60.051099059926763  ActiveDisplayYMaximum=540.45256909803  DataLoggingVariableName=ScopeData29
  wires:
  [mosfet_voltage_invQ1] -> mosfet power losses INV Q1/2  "mosfet_voltage_invQ1"
  [mosfet_current_invQ2] -> mosfet power losses INV Q2/3  "mosfet_current_invQ2"
  [mosfet_ploss_invQ1] -> mosfet power losses INV Q1/1  "mosfet_ploss_invQ1"
  [mosfet_ploss_invQ2] -> mosfet power losses INV Q2/1  "mosfet_ploss_invQ2"
  [mosfet_JH_temp_invQ2] -> Bus Creator9/1  "mosfet_JH_temp_invQ2"
  [mosfet_HA_temp_invQ1] -> Bus Creator8/2  "mosfet_HA_temp_invQ1"
  [mosfet_current_invQ1] -> mosfet power losses INV Q1/3  "mosfet_current_invQ1"
  [mosfet_JH_temp_invQ1] -> Bus Creator8/1  "mosfet_JH_temp_invQ1"
  [mosfet_HA_temp_invQ2] -> Bus Creator9/2  "mosfet_HA_temp_invQ2"
  [mosfet_voltage_invQ2] -> mosfet power losses INV Q2/2  "mosfet_voltage_invQ2"
  Bus Creator8/1 -> mosfet power losses INV Q1/4
  Bus Creator9/1 -> mosfet power losses INV Q2/4

== system inv_psm/inv_psm_mod1/inverter/inverter ==
  gate_cmds_uvw : Inport
  sv_pwm : Subsystem
  three_phase_inverter_ideal_switch_based_model : Subsystem
  three_phase_inverter_igbt_adv_thermal_model : Subsystem  Commented=on
  three_phase_inverter_mosfet_based_with_thermal_model : Subsystem  Commented=on
  u : PMIOPort  Side=Left
  v : PMIOPort  Port=2  Side=Left
  w : PMIOPort  Port=3  Side=Left
  udc(+) : PMIOPort  Port=4  Side=Right
  udc(-) : PMIOPort  Port=5  Side=Right
  wires:
  sv_pwm/1(gate_cmds) -> three_phase_inverter_mosfet_based_with_thermal_model/1(gate_commands), three_phase_inverter_igbt_adv_thermal_model/1(gate_commands), three_phase_inverter_ideal_switch_based_model/1(gate_commands)
  gate_cmds_uvw/1 -> sv_pwm/1(gate_cmds_uvw)
  connections:
  udc(+)/RConn1 -- three_phase_inverter_igbt_adv_thermal_model/LConn1 -- three_phase_inverter_mosfet_based_with_thermal_model/LConn1 -- three_phase_inverter_ideal_switch_based_model/LConn1
  u/RConn1 -- three_phase_inverter_igbt_adv_thermal_model/RConn1 -- three_phase_inverter_ideal_switch_based_model/RConn1 -- three_phase_inverter_mosfet_based_with_thermal_model/RConn1
  v/RConn1 -- three_phase_inverter_igbt_adv_thermal_model/RConn2 -- three_phase_inverter_ideal_switch_based_model/RConn2 -- three_phase_inverter_mosfet_based_with_thermal_model/RConn2
  w/RConn1 -- three_phase_inverter_igbt_adv_thermal_model/RConn3 -- three_phase_inverter_ideal_switch_based_model/RConn3 -- three_phase_inverter_mosfet_based_with_thermal_model/RConn3
  three_phase_inverter_mosfet_based_with_thermal_model/LConn2 -- three_phase_inverter_igbt_adv_thermal_model/LConn2 -- udc(-)/RConn1 -- three_phase_inverter_ideal_switch_based_model/LConn2

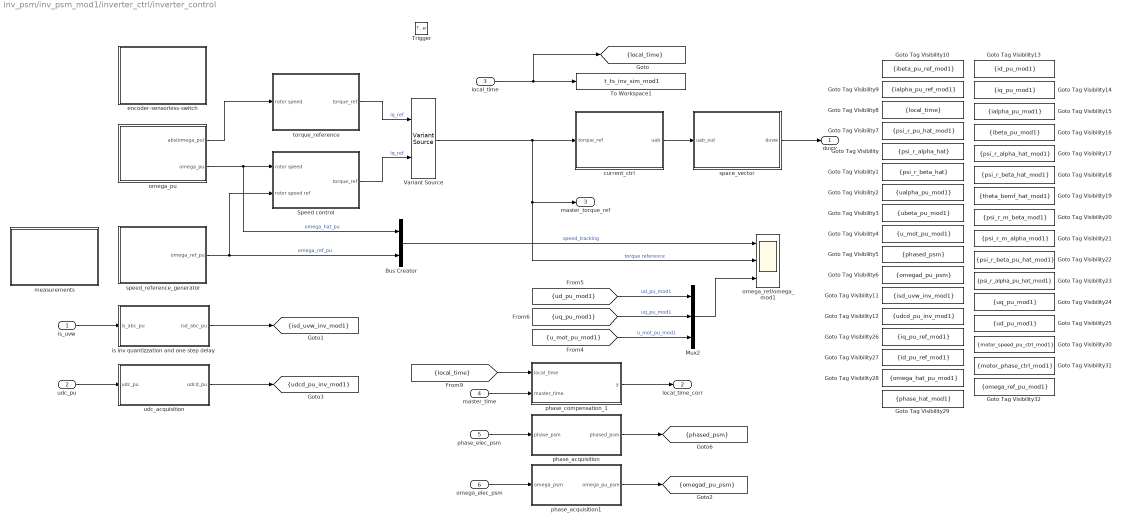
== system inv_psm/inv_psm_mod1/inverter_ctrl/inverter_control ==
  is_uvw : Inport
  udc_pu : Inport  Port=2
  local_time : Inport  Port=3
  master_time : Inport  Port=4
  phase_elec_psm : Inport  Port=5
  omega_elec_psm : Inport  Port=6
  Trigger : TriggerPort  VariantControl=(inherit)  PortDimensions=1
  Bus Creator : BusCreator  Inputs=2
  Goto Tag Visibility : GotoTagVisibility  GotoTag=psi_r_alpha_hat
  Goto Tag Visibility1 : GotoTagVisibility  GotoTag=psi_r_beta_hat
  Goto Tag Visibility10 : GotoTagVisibility  GotoTag=ibeta_pu_ref_mod1
  Goto Tag Visibility11 : GotoTagVisibility  GotoTag=isd_uvw_inv_mod1
  Goto Tag Visibility12 : GotoTagVisibility  GotoTag=udcd_pu_inv_mod1
  Goto Tag Visibility13 : GotoTagVisibility  GotoTag=id_pu_mod1
  Goto Tag Visibility14 : GotoTagVisibility  GotoTag=iq_pu_mod1
  Goto Tag Visibility15 : GotoTagVisibility  GotoTag=ialpha_pu_mod1
  Goto Tag Visibility16 : GotoTagVisibility  GotoTag=ibeta_pu_mod1
  Goto Tag Visibility17 : GotoTagVisibility  GotoTag=psi_r_alpha_hat_mod1
  Goto Tag Visibility18 : GotoTagVisibility  GotoTag=psi_r_beta_hat_mod1
  Goto Tag Visibility19 : GotoTagVisibility  GotoTag=theta_bemf_hat_mod1
  Goto Tag Visibility2 : GotoTagVisibility  GotoTag=ualpha_pu_mod1
  Goto Tag Visibility20 : GotoTagVisibility  GotoTag=psi_r_m_beta_mod1
  Goto Tag Visibility21 : GotoTagVisibility  GotoTag=psi_r_m_alpha_mod1
  Goto Tag Visibility22 : GotoTagVisibility  GotoTag=psi_r_beta_pu_hat_mod1
  Goto Tag Visibility23 : GotoTagVisibility  GotoTag=psi_r_alpha_pu_hat_mod1
  Goto Tag Visibility24 : GotoTagVisibility  GotoTag=uq_pu_mod1
  Goto Tag Visibility25 : GotoTagVisibility  GotoTag=ud_pu_mod1
  Goto Tag Visibility26 : GotoTagVisibility  GotoTag=iq_pu_ref_mod1
  Goto Tag Visibility27 : GotoTagVisibility  GotoTag=id_pu_ref_mod1
  Goto Tag Visibility28 : GotoTagVisibility  GotoTag=omega_hat_pu_mod1
  Goto Tag Visibility29 : GotoTagVisibility  GotoTag=phase_hat_mod1
  Goto Tag Visibility3 : GotoTagVisibility  GotoTag=ubeta_pu_mod1
  Goto Tag Visibility30 : GotoTagVisibility  GotoTag=motor_speed_pu_ctrl_mod1
  Goto Tag Visibility31 : GotoTagVisibility  GotoTag=motor_phase_ctrl_mod1
  Goto Tag Visibility32 : GotoTagVisibility  GotoTag=omega_ref_pu_mod1
  Goto Tag Visibility4 : GotoTagVisibility  GotoTag=u_mot_pu_mod1
  Goto Tag Visibility5 : GotoTagVisibility  GotoTag=phased_psm
  Goto Tag Visibility6 : GotoTagVisibility  GotoTag=omegad_pu_psm
  Goto Tag Visibility7 : GotoTagVisibility  GotoTag=psi_r_pu_hat_mod1
  Goto Tag Visibility8 : GotoTagVisibility  GotoTag=local_time
  Goto Tag Visibility9 : GotoTagVisibility  GotoTag=ialpha_pu_ref_mod1
  Mux2 : Mux  Inputs=3
  Speed control : Subsystem
  To Workspace1 : ToWorkspace  VariableName=t_ts_inv_sim_mod1  SampleTime=-1
      settings: MaxDataPoints=param.glb_time.Ns_inv
  Variant Source : VariantSource  VariantControls={param.psm.mode.use_torque_curve == 1, param.psm.mode.use_speed_control == 1}
  current_ctrl : Subsystem
  encoder-sensorless-switch : Subsystem
  is inv quantizzation and one step delay : Subsystem
  measurements : Subsystem
  omega_pu : Subsystem
  omega_ref/omega_mod1 : Scope  NumInputPorts=3
      settings: ActiveDisplayYMinimum=-0.12532671338506449  ActiveDisplayYMaximum=1.1279404204655807  DataLoggingVariableName=ScopeData3
  phase_acquisition : Subsystem
  phase_acquisition1 : Subsystem
  phase_compensation_1 : Subsystem
  space_vector : Subsystem
  speed_reference_generator : Subsystem
  torque_reference : Subsystem
  udc_acquisition : Subsystem
  duvw : Outport  VectorParamsAs1DForOutWhenUnconnected=off
  local_time_corr : Outport  Port=2
  master_torque_ref : Outport  Port=3  VectorParamsAs1DForOutWhenUnconnected=off
  tag scope: isd_uvw_inv_mod1=scoped, local_time=scoped, omegad_pu_psm=scoped, phased_psm=scoped, udcd_pu_inv_mod1=scoped
  wires:
  speed_reference_generator/1(omega_ref_pu) -> Speed control/2(rotor speed ref), Bus Creator/2  "omega_ref_pu"
  Bus Creator/1 -> omega_ref/omega_mod1/1  "speed_tracking"
  Variant Source/1 -> current_ctrl/1(torque_ref), master_torque_ref/1, omega_ref/omega_mod1/2  "torque reference"
  [ud_pu_mod1] -> Mux2/1  "ud_pu_mod1"
  [uq_pu_mod1] -> Mux2/2  "uq_pu_mod1"
  Mux2/1 -> omega_ref/omega_mod1/3
  [u_mot_pu_mod1] -> Mux2/3  "u_mot_pu_mod1"
  omega_pu/2(omega_pu) -> Bus Creator/1, Speed control/1(rotor speed)  "omega_hat_pu"
  omega_pu/1(abs(omega_pu)) -> torque_reference/1(rotor speed)
  torque_reference/1(torque_ref) -> Variant Source/1  "iq_ref"
  Speed control/1(torque_ref) -> Variant Source/2  "iq_ref"
  udc_acquisition/1(udcd_pu) -> [udcd_pu_inv_mod1]
  udc_pu/1 -> udc_acquisition/1(udc_pu)
  is_uvw/1 -> is inv quantizzation and one step delay/1(is_abc_pu)
  is inv quantizzation and one step delay/1(isd_abc_pu) -> [isd_uvw_inv_mod1]
  local_time/1 -> To Workspace1/1, [local_time]
  current_ctrl/1(uab) -> space_vector/1(uab_out)
  space_vector/1(duvw) -> duvw/1
  master_time/1 -> phase_compensation_1/2(master_time)
  [local_time] -> phase_compensation_1/1(local_time)
  phase_compensation_1/1(y) -> local_time_corr/1
  phase_acquisition/1(phased_psm) -> [phased_psm]
  phase_elec_psm/1 -> phase_acquisition/1(phase_psm)
  omega_elec_psm/1 -> phase_acquisition1/1(omega_psm)
  phase_acquisition1/1(omega_pu_psm) -> [omegad_pu_psm]
